simulink model "gm_PMLSM_FOC_FixedPoint_vnl"  (R2026b)
settings: Solver=FixedStepDiscrete  StopTime=0.0063  FixedStep=2e-08
undefined symbols (not defined in the file): FOC_Fixed_Config, Lookup, Ts_ACR
libraries: hdlmdlgenlib x38, simulink x16, mcbeeMathTransformLib x2
(part 6 of 6)

== system gm_PMLSM_FOC_FixedPoint_vnl/FOC_DUT/FOC_DUT/InversePark/Variant/mcb/Inverse Park Transform/Select/Two Inputs/Two inputs CRL ==
  D : Inport  OutDataTypeStr=fixdt(1, 64, 40)  PortDimensions=1  SampleTime=2e-08
  Q : Inport  Port=2  OutDataTypeStr=fixdt(1, 64, 40)  PortDimensions=1  SampleTime=2e-08
  sin : Inport  Port=3  OutDataTypeStr=fixdt(1, 40, 32)  PortDimensions=1  SampleTime=2e-08
  cos : Inport  Port=4  OutDataTypeStr=fixdt(1, 40, 32)  PortDimensions=1  SampleTime=2e-08
  Switch_Axis : Subsystem
  dcos : Product  Inputs=**  OutDataTypeStr=fixdt(1, 104, 72)  SampleTime=2e-08
  dcos_out_dtc : DataTypeConversion  OutDataTypeStr=fixdt(1, 64, 40)  RndMeth=Simplest  SampleTime=2e-08  SaturateOnIntegerOverflow=off
  dsin : Product  Inputs=**  OutDataTypeStr=fixdt(1, 104, 72)  SampleTime=2e-08
  dsin_out_dtc : DataTypeConversion  OutDataTypeStr=fixdt(1, 64, 40)  RndMeth=Simplest  SampleTime=2e-08  SaturateOnIntegerOverflow=off
  qcos : Product  Inputs=**  OutDataTypeStr=fixdt(1, 104, 72)  SampleTime=2e-08
  qcos_out_dtc : DataTypeConversion  OutDataTypeStr=fixdt(1, 64, 40)  RndMeth=Simplest  SampleTime=2e-08  SaturateOnIntegerOverflow=off
  qsin : Product  Inputs=**  OutDataTypeStr=fixdt(1, 104, 72)  SampleTime=2e-08
  qsin_out_dtc : DataTypeConversion  OutDataTypeStr=fixdt(1, 64, 40)  RndMeth=Simplest  SampleTime=2e-08  SaturateOnIntegerOverflow=off
  rd_0 : Delay  DelayLength=162  InitialCondition=0  SampleTime=2e-08
  rd_1 : Delay  DelayLength=162  InitialCondition=0  SampleTime=2e-08
  rd_{2..5} (4 alike) : Delay  DelayLength=1  InitialCondition=0  SampleTime=2e-08
  sum_alpha : Sum  Inputs=+-  OutDataTypeStr=fixdt(1, 64, 40)  AccumDataTypeStr=fixdt(1, 64, 40)  RndMeth=Simplest  SampleTime=2e-08
  sum_beta : Sum  OutDataTypeStr=fixdt(1, 64, 40)  AccumDataTypeStr=fixdt(1, 64, 40)  RndMeth=Simplest  SampleTime=2e-08
  AlphaO : Outport  OutDataTypeStr=fixdt(1, 64, 40)  PortDimensions=1  SampleTime=2e-08  VectorParamsAs1DForOutWhenUnconnected=off
  BetaO : Outport  Port=2  OutDataTypeStr=fixdt(1, 64, 40)  PortDimensions=1  SampleTime=2e-08  VectorParamsAs1DForOutWhenUnconnected=off
  wires:
  Switch_Axis/1(Alpha) -> AlphaO/1
  dsin_out_dtc/1 -> sum_beta/2
  qcos_out_dtc/1 -> sum_beta/1
  qsin_out_dtc/1 -> sum_alpha/2
  dcos_out_dtc/1 -> sum_alpha/1
  rd_5/1 -> dsin_out_dtc/1
  rd_4/1 -> qcos_out_dtc/1
  rd_3/1 -> qsin_out_dtc/1
  rd_2/1 -> dcos_out_dtc/1
  dsin/1 -> rd_5/1
  sum_beta/1 -> Switch_Axis/2(B)
  qcos/1 -> rd_4/1
  Switch_Axis/2(Beta) -> BetaO/1
  dcos/1 -> rd_2/1
  sum_alpha/1 -> Switch_Axis/1(A)
  rd_0/1 -> qcos/2, dcos/2
  Q/1 -> qcos/1, qsin/1
  D/1 -> dcos/1, dsin/1
  sin/1 -> rd_1/1
  rd_1/1 -> qsin/2, dsin/2
  qsin/1 -> rd_3/1
  cos/1 -> rd_0/1

== system gm_PMLSM_FOC_FixedPoint_vnl/FOC_DUT/FOC_DUT/InversePark/Variant/mcb/sinecos/Sine-Cosine Lookup/WrapUp/If Action Subsystem ==
  In1 : Inport  OutDataTypeStr=fixdt(1, 40, 32)  PortDimensions=1  SampleTime=0.0001
  Action Port : Inport  Port=2  OutDataTypeStr=boolean  PortDimensions=1  SampleTime=0.0001
  Convert_back : DataTypeConversion  OutDataTypeStr=fixdt(1, 40, 32)  RndMeth=Simplest  SampleTime=0.0001  SaturateOnIntegerOverflow=off
  Convert_uint16 : DataTypeConversion  OutDataTypeStr=int16  SampleTime=0.0001  SaturateOnIntegerOverflow=off  RndMeth=Floor
  Out1_bypass : UnitDelay  InitialCondition="fi(0,1,40,32,\"hex\",\"0000000000\")"  SampleTime=0.0001
  Sum : Sum  Inputs=+-  OutDataTypeStr=fixdt(1, 40, 32)  AccumDataTypeStr=fixdt(1, 40, 32)  RndMeth=Simplest  SampleTime=0.0001
  Sum_out1bypassMux : Switch  Criteria=u2 ~= 0  OutDataTypeStr=fixdt(1, 40, 32)  SampleTime=0.0001  SaturateOnIntegerOverflow=off  InputSameDT=off
  Out1 : Outport  OutDataTypeStr=fixdt(1, 40, 32)  PortDimensions=1  SampleTime=0.0001  InitialOutput=0
  wires:
  Out1_bypass/1 -> Sum_out1bypassMux/3
  Sum_out1bypassMux/1 -> Out1_bypass/1, Out1/1
  Convert_back/1 -> Sum/2
  Convert_uint16/1 -> Convert_back/1
  Action Port/1 -> Sum_out1bypassMux/2
  In1/1 -> Convert_uint16/1, Sum/1
  Sum/1 -> Sum_out1bypassMux/1

== system gm_PMLSM_FOC_FixedPoint_vnl/FOC_DUT/FOC_DUT/InversePark/Variant/mcb/sinecos/Sine-Cosine Lookup/WrapUp/If Action Subsystem1 ==
  In1 : Inport  OutDataTypeStr=fixdt(1, 40, 32)  PortDimensions=1  SampleTime=0.0001
  Action Port : Inport  Port=2  OutDataTypeStr=boolean  PortDimensions=1  SampleTime=0.0001
  Convert_back : DataTypeConversion  OutDataTypeStr=fixdt(1, 40, 32)  RndMeth=Simplest  SampleTime=0.0001  SaturateOnIntegerOverflow=off
  Convert_uint16 : DataTypeConversion  OutDataTypeStr=int16  RndMeth=Simplest  SampleTime=0.0001  SaturateOnIntegerOverflow=off
  Out1_bypass : UnitDelay  InitialCondition="fi(0,1,40,32,\"hex\",\"0000000000\")"  SampleTime=0.0001
  Sum : Sum  Inputs=+-  OutDataTypeStr=fixdt(1, 40, 32)  AccumDataTypeStr=fixdt(1, 40, 32)  RndMeth=Simplest  SampleTime=0.0001
  Sum_out1bypassMux : Switch  Criteria=u2 ~= 0  OutDataTypeStr=fixdt(1, 40, 32)  SampleTime=0.0001  SaturateOnIntegerOverflow=off  InputSameDT=off
  Out1 : Outport  OutDataTypeStr=fixdt(1, 40, 32)  PortDimensions=1  SampleTime=0.0001  InitialOutput=0
  wires:
  Sum_out1bypassMux/1 -> Out1/1, Out1_bypass/1
  Sum/1 -> Sum_out1bypassMux/1
  Convert_back/1 -> Sum/2
  Convert_uint16/1 -> Convert_back/1
  Action Port/1 -> Sum_out1bypassMux/2
  In1/1 -> Convert_uint16/1, Sum/1
  Out1_bypass/1 -> Sum_out1bypassMux/3

== system gm_PMLSM_FOC_FixedPoint_vnl/FOC_DUT/FOC_DUT/InversePark/Variant/mcb/sinecos/Sine-Cosine Lookup/datatype/datatype no change ==
  In1 : Inport  OutDataTypeStr=fixdt(1, 40, 32)  PortDimensions=[4]  SampleTime=2e-08
  Out1 : Outport  OutDataTypeStr=fixdt(1, 40, 32)  PortDimensions=[4]  SampleTime=2e-08
  wires:
  In1/1 -> Out1/1

== system gm_PMLSM_FOC_FixedPoint_vnl/FOC_DUT/FOC_DUT/Park/Variant/mcb/Park Transform/Select/Two Inputs/Two inputs CRL ==
  AlphaIn : Inport  OutDataTypeStr=fixdt(1, 64, 40)  PortDimensions=1  SampleTime=0.0001
  BetaIn : Inport  Port=2  OutDataTypeStr=fixdt(1, 64, 40)  PortDimensions=1  SampleTime=0.0001
  sine : Inport  Port=3  OutDataTypeStr=fixdt(1, 40, 32)  PortDimensions=1  SampleTime=0.0001
  cos : Inport  Port=4  OutDataTypeStr=fixdt(1, 40, 32)  PortDimensions=1  SampleTime=0.0001
  Switch_Axis : Subsystem
  acos : Product  Inputs=**  OutDataTypeStr=fixdt(1, 104, 72)  SampleTime=0.0001
  acos_out_dtc : DataTypeConversion  OutDataTypeStr=fixdt(1, 64, 40)  RndMeth=Simplest  SampleTime=0.0001  SaturateOnIntegerOverflow=off
  asin : Product  Inputs=**  OutDataTypeStr=fixdt(1, 104, 72)  SampleTime=0.0001
  asin_out_dtc : DataTypeConversion  OutDataTypeStr=fixdt(1, 64, 40)  RndMeth=Simplest  SampleTime=0.0001  SaturateOnIntegerOverflow=off
  bcos : Product  Inputs=**  OutDataTypeStr=fixdt(1, 104, 72)  SampleTime=0.0001
  bcos_out_dtc : DataTypeConversion  OutDataTypeStr=fixdt(1, 64, 40)  RndMeth=Simplest  SampleTime=0.0001  SaturateOnIntegerOverflow=off
  bsin : Product  Inputs=**  OutDataTypeStr=fixdt(1, 104, 72)  SampleTime=0.0001
  bsin_out_dtc : DataTypeConversion  OutDataTypeStr=fixdt(1, 64, 40)  RndMeth=Simplest  SampleTime=0.0001  SaturateOnIntegerOverflow=off
  sum_Ds : Sum  OutDataTypeStr=fixdt(1, 64, 40)  AccumDataTypeStr=fixdt(1, 64, 40)  RndMeth=Simplest  SampleTime=0.0001
  sum_Qs : Sum  Inputs=+-  OutDataTypeStr=fixdt(1, 64, 40)  AccumDataTypeStr=fixdt(1, 64, 40)  RndMeth=Simplest  SampleTime=0.0001
  D : Outport  OutDataTypeStr=fixdt(1, 64, 40)  PortDimensions=1  SampleTime=0.0001  VectorParamsAs1DForOutWhenUnconnected=off
  Q : Outport  Port=2  OutDataTypeStr=fixdt(1, 64, 40)  PortDimensions=1  SampleTime=0.0001  VectorParamsAs1DForOutWhenUnconnected=off
  wires:
  Switch_Axis/1(d_axis) -> D/1
  Switch_Axis/2(q_axis) -> Q/1
  sum_Qs/1 -> Switch_Axis/2(q)
  sum_Ds/1 -> Switch_Axis/1(d)
  bcos_out_dtc/1 -> sum_Qs/1
  asin_out_dtc/1 -> sum_Qs/2
  bsin_out_dtc/1 -> sum_Ds/2
  acos_out_dtc/1 -> sum_Ds/1
  asin/1 -> asin_out_dtc/1
  acos/1 -> acos_out_dtc/1
  bsin/1 -> bsin_out_dtc/1
  BetaIn/1 -> bcos/1, bsin/1
  sine/1 -> asin/2, bsin/2
  cos/1 -> acos/2, bcos/2
  bcos/1 -> bcos_out_dtc/1
  AlphaIn/1 -> acos/1, asin/1

== system gm_PMLSM_FOC_FixedPoint_vnl/FOC_DUT/FOC_DUT/Park/Variant/mcb/sinecos/Sine-Cosine Lookup/WrapUp/If Action Subsystem ==
  In1 : Inport  OutDataTypeStr=fixdt(1, 40, 32)  PortDimensions=1  SampleTime=0.0001
  Action Port : Inport  Port=2  OutDataTypeStr=boolean  PortDimensions=1  SampleTime=0.0001
  Convert_back : DataTypeConversion  OutDataTypeStr=fixdt(1, 40, 32)  RndMeth=Simplest  SampleTime=0.0001  SaturateOnIntegerOverflow=off
  Convert_uint16 : DataTypeConversion  OutDataTypeStr=int16  SampleTime=0.0001  SaturateOnIntegerOverflow=off  RndMeth=Floor
  Out1_bypass : UnitDelay  InitialCondition="fi(0,1,40,32,\"hex\",\"0000000000\")"  SampleTime=0.0001
  Sum : Sum  Inputs=+-  OutDataTypeStr=fixdt(1, 40, 32)  AccumDataTypeStr=fixdt(1, 40, 32)  RndMeth=Simplest  SampleTime=0.0001
  Sum_out1bypassMux : Switch  Criteria=u2 ~= 0  OutDataTypeStr=fixdt(1, 40, 32)  SampleTime=0.0001  SaturateOnIntegerOverflow=off  InputSameDT=off
  Out1 : Outport  OutDataTypeStr=fixdt(1, 40, 32)  PortDimensions=1  SampleTime=0.0001  InitialOutput=0
  wires:
  Sum/1 -> Sum_out1bypassMux/1
  In1/1 -> Sum/1, Convert_uint16/1
  Action Port/1 -> Sum_out1bypassMux/2
  Convert_uint16/1 -> Convert_back/1
  Convert_back/1 -> Sum/2
  Sum_out1bypassMux/1 -> Out1/1, Out1_bypass/1
  Out1_bypass/1 -> Sum_out1bypassMux/3

== system gm_PMLSM_FOC_FixedPoint_vnl/FOC_DUT/FOC_DUT/Park/Variant/mcb/sinecos/Sine-Cosine Lookup/WrapUp/If Action Subsystem1 ==
  In1 : Inport  OutDataTypeStr=fixdt(1, 40, 32)  PortDimensions=1  SampleTime=0.0001
  Action Port : Inport  Port=2  OutDataTypeStr=boolean  PortDimensions=1  SampleTime=0.0001
  Convert_back : DataTypeConversion  OutDataTypeStr=fixdt(1, 40, 32)  RndMeth=Simplest  SampleTime=0.0001  SaturateOnIntegerOverflow=off
  Convert_uint16 : DataTypeConversion  OutDataTypeStr=int16  RndMeth=Simplest  SampleTime=0.0001  SaturateOnIntegerOverflow=off
  Out1_bypass : UnitDelay  InitialCondition="fi(0,1,40,32,\"hex\",\"0000000000\")"  SampleTime=0.0001
  Sum : Sum  Inputs=+-  OutDataTypeStr=fixdt(1, 40, 32)  AccumDataTypeStr=fixdt(1, 40, 32)  RndMeth=Simplest  SampleTime=0.0001
  Sum_out1bypassMux : Switch  Criteria=u2 ~= 0  OutDataTypeStr=fixdt(1, 40, 32)  SampleTime=0.0001  SaturateOnIntegerOverflow=off  InputSameDT=off
  Out1 : Outport  OutDataTypeStr=fixdt(1, 40, 32)  PortDimensions=1  SampleTime=0.0001  InitialOutput=0
  wires:
  Out1_bypass/1 -> Sum_out1bypassMux/3
  In1/1 -> Sum/1, Convert_uint16/1
  Action Port/1 -> Sum_out1bypassMux/2
  Convert_uint16/1 -> Convert_back/1
  Convert_back/1 -> Sum/2
  Sum/1 -> Sum_out1bypassMux/1
  Sum_out1bypassMux/1 -> Out1_bypass/1, Out1/1

== system gm_PMLSM_FOC_FixedPoint_vnl/FOC_DUT/FOC_DUT/Park/Variant/mcb/sinecos/Sine-Cosine Lookup/datatype/datatype no change ==
  In1 : Inport  OutDataTypeStr=fixdt(1, 40, 32)  PortDimensions=[4]  SampleTime=0.0001
  Out1 : Outport  OutDataTypeStr=fixdt(1, 40, 32)  PortDimensions=[4]  SampleTime=0.0001
  wires:
  In1/1 -> Out1/1

== system gm_PMLSM_FOC_FixedPoint_vnl/FOC_DUT/FOC_DUT/InversePark/Variant/mcb/Inverse Park Transform/Select/Two Inputs/Two inputs CRL/Switch_Axis ==
  A : Inport  OutDataTypeStr=fixdt(1, 64, 40)  PortDimensions=1  SampleTime=2e-08
  B : Inport  Port=2  OutDataTypeStr=fixdt(1, 64, 40)  PortDimensions=1  SampleTime=2e-08
  Offset : Constant  Value=0  OutDataTypeStr=uint16  SampleTime=2e-08
  Switch : Switch  Criteria=u2 > Threshold  Threshold="fi(0,0,16,0,\"hex\",\"0001\")"  OutDataTypeStr=fixdt(1, 64, 40)  RndMeth=Simplest  SampleTime=2e-08  SaturateOnIntegerOverflow=off  InputSameDT=off
  Unary_Minus : UnaryMinus  SampleTime=2e-08
  delayMatch : Delay  DelayLength=1  InitialCondition=0  SampleTime=2e-08
  delayMatch1 : Delay  DelayLength=1  InitialCondition=0  SampleTime=2e-08
  mux : Mux  Inputs=2
  mux1 : Mux  Inputs=2
  t : Demux  Outputs=2
  Alpha : Outport  OutDataTypeStr=fixdt(1, 64, 40)  PortDimensions=1  SampleTime=2e-08  VectorParamsAs1DForOutWhenUnconnected=off
  Beta : Outport  Port=2  OutDataTypeStr=fixdt(1, 64, 40)  PortDimensions=1  SampleTime=2e-08  VectorParamsAs1DForOutWhenUnconnected=off
  wires:
  t/1 -> Alpha/1
  t/2 -> Beta/1
  Switch/1 -> t/1
  mux/1 -> Switch/3
  Offset/1 -> Switch/2
  mux1/1 -> Switch/1
  delayMatch1/1 -> mux1/1, mux/2
  B/1 -> delayMatch1/1
  delayMatch/1 -> Unary_Minus/1, mux/1
  A/1 -> delayMatch/1
  Unary_Minus/1 -> mux1/2

== system gm_PMLSM_FOC_FixedPoint_vnl/FOC_DUT/FOC_DUT/Park/Variant/mcb/Park Transform/Select/Two Inputs/Two inputs CRL/Switch_Axis ==
  d : Inport  OutDataTypeStr=fixdt(1, 64, 40)  PortDimensions=1  SampleTime=0.0001
  q : Inport  Port=2  OutDataTypeStr=fixdt(1, 64, 40)  PortDimensions=1  SampleTime=0.0001
  Offset : Constant  Value=0  OutDataTypeStr=uint16  SampleTime=0.0001
  Switch : Switch  Criteria=u2 > Threshold  Threshold="fi(0,0,16,0,\"hex\",\"0001\")"  OutDataTypeStr=fixdt(1, 64, 40)  RndMeth=Simplest  SampleTime=0.0001  SaturateOnIntegerOverflow=off  InputSameDT=off
  Unary_Minus : UnaryMinus  SampleTime=0.0001
  mux : Mux  Inputs=2
  mux1 : Mux  Inputs=2
  t : Demux  Outputs=2
  d_axis : Outport  OutDataTypeStr=fixdt(1, 64, 40)  PortDimensions=1  SampleTime=0.0001  VectorParamsAs1DForOutWhenUnconnected=off
  q_axis : Outport  Port=2  OutDataTypeStr=fixdt(1, 64, 40)  PortDimensions=1  SampleTime=0.0001  VectorParamsAs1DForOutWhenUnconnected=off
  wires:
  t/1 -> d_axis/1
  t/2 -> q_axis/1
  Switch/1 -> t/1
  mux/1 -> Switch/3
  Offset/1 -> Switch/2
  mux1/1 -> Switch/1
  Unary_Minus/1 -> mux1/1
  d/1 -> mux/1, mux1/2
  q/1 -> Unary_Minus/1, mux/2
